simulink model "DynamicsHIL"  (R2026a)
settings: Solver=ode4  StopTime=inf  FixedStep=SampleTime
values from neighbouring files (symbols this model uses):
  ArmConstants = struct('l1_dim', l1_dim,                        'l2_dim', l2_dim,                        'Hexa_to_joint_L', L,                        'Mass1', ml1,                        'Mass2', ml2,                        'Inertia1', Hl1,                        'Inertia2', Hl2,                        'MC1', c1,                        'MC2', c2,                        'Servos', Servos)    [init_model.m]    (also in init_var.m)
  HexaConstants = struct('Mass', mb,                         'Inertia', J ,                         'allo', allo,                          'invallo', invallo,                         'kT', kT)    [init_model.m]    (also in init_var.m)
  SampleTime = 0.01    [init_model.m]    (also in px4HostTarget_TCPIP_Read.m = -1)
undefined symbols (not defined in the file or in its folder): Payload
libraries: uavmavlinklib x3, px4MAVLinkBridgelib x2
settings Model: Creator=The MathWorks, Inc.  LastModifiedBy=Carlos Fabian

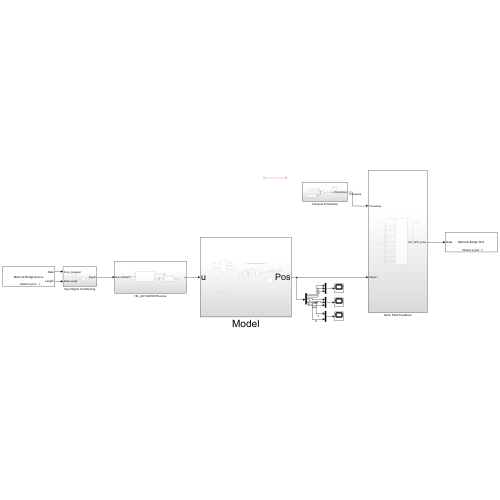
[thumbnail: Simulink's stored preview of the top-level diagram]
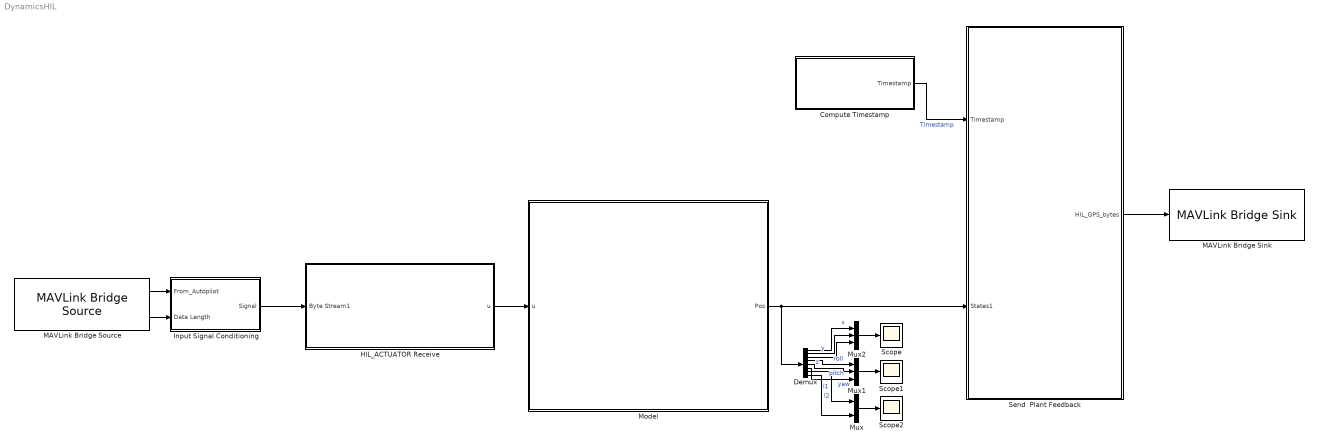
== system DynamicsHIL ==
  Compute Timestamp : Subsystem
  Demux : Demux  Outputs=8
  HIL_ACTUATOR Receive : Subsystem
  Input Signal Conditioning : Subsystem
  MAVLink Bridge Sink : px4MAVLinkBridgelib/MAVLink Bridge Sink  PixhawkSerialPorttemp=<Select a port...>  PixhawkSerialPortManually=COM12  FieldTable={ 'UDP', '127.0.0.1', '14550' }
  MAVLink Bridge Source : px4MAVLinkBridgelib/MAVLink Bridge Source  PixhawkSerialPorttemp=<Select a port...>  PixhawkSerialPortManually=COM12  dataLength=MAVLink_Input_Read_Size  FieldTable={ 'UDP', '127.0.0.1', '14550' }  SampleTime=SampleTime
  Model : Subsystem
  Mux : Mux  Inputs=2
  Mux1 : Mux  Inputs=3
  Mux2 : Mux  Inputs=3
  Scope : Scope
  Scope1 : Scope
  Scope2 : Scope
      settings: DataLoggingVariableName=ScopeData2
  Send  Plant Feedback : Subsystem
  wires:
  ? -> ?
  Input Signal Conditioning/1(Signal) -> HIL_ACTUATOR Receive/1(Byte Stream1)
  MAVLink Bridge Source/1 -> Input Signal Conditioning/1(From_Autopilot)
  MAVLink Bridge Source/2 -> Input Signal Conditioning/2(Data Length)
  Send  Plant Feedback/1(HIL_GPS_bytes) -> MAVLink Bridge Sink/1
  Compute Timestamp/1(Timestamp) -> Send  Plant Feedback/1(Timestamp)  "Timestamp"
  Model/1(Pos) -> Demux/1, Send  Plant Feedback/2(States1)
  HIL_ACTUATOR Receive/1(u) -> Model/1(u)
  Demux/1 -> Mux2/1  "x"
  Demux/2 -> Mux2/2  "y"
  Demux/3 -> Mux2/3  "z"
  Demux/4 -> Mux1/1  "roll"
  Demux/5 -> Mux1/2  "pitch"
  Demux/6 -> Mux1/3  "yaw"
  Demux/8 -> Mux/2  "l2"
  Demux/7 -> Mux/1  "l1"
  Mux2/1 -> Scope/1
  Mux1/1 -> Scope1/1
  Mux/1 -> Scope2/1

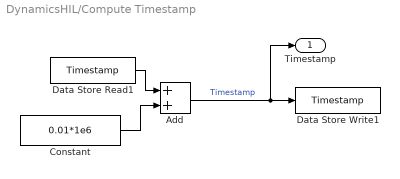
== system DynamicsHIL/Compute Timestamp ==
  Add : Sum
  Constant : Constant  Value=0.01*1e6  OutDataTypeStr=uint64  SampleTime=0.01
  Data Store Read1 : DataStoreRead  DataStoreName=Timestamp  SampleTime=0.01  IndexOptions=Index vector (dialog)  Indices=1  OutputSizes=1
  Data Store Write1 : DataStoreWrite  DataStoreName=Timestamp  SampleTime=0.01  IndexOptions=Index vector (dialog)  Indices=1  OutputSizes=1
  Timestamp : Outport
  wires:
  Data Store Read1/1 -> Add/1
  Add/1 -> Data Store Write1/1, Timestamp/1  "Timestamp"
  Constant/1 -> Add/2

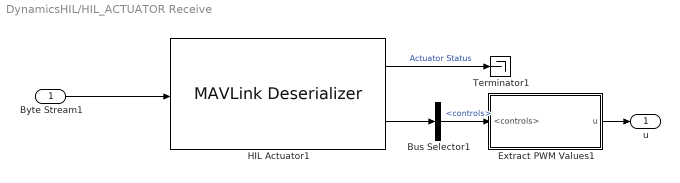
== system DynamicsHIL/HIL_ACTUATOR Receive ==
  Byte Stream1 : Inport
  Bus Selector1 : BusSelector  OutputSignals=Payload.controls
  Extract PWM Values1 : Subsystem
  HIL Actuator1 : uavmavlinklib/MAVLink Deserializer  dialectSource=Specify your own  dialect=common.xml  dialectCustom=C:\Users\Carlos Fabian\Documents\MATLAB\mavlink_custom\uam.xml  version=2  messageType=HIL_ACTUATOR_CONTROLS  inputDataLength=off  SystemIDFilter=off  systemID=1  ComponentIDFilter=off  componentID=1  queueMsg=off  queueMsgSize=50  dropNum=off
  Terminator1 : Terminator
  u : Outport
  wires:
  HIL Actuator1/2 -> Bus Selector1/1
  HIL Actuator1/1 -> Terminator1/1  "Actuator Status"
  Extract PWM Values1/1(u) -> u/1
  Bus Selector1/1 -> Extract PWM Values1/1(<controls>)  "<controls>"
  Byte Stream1/1 -> HIL Actuator1/1

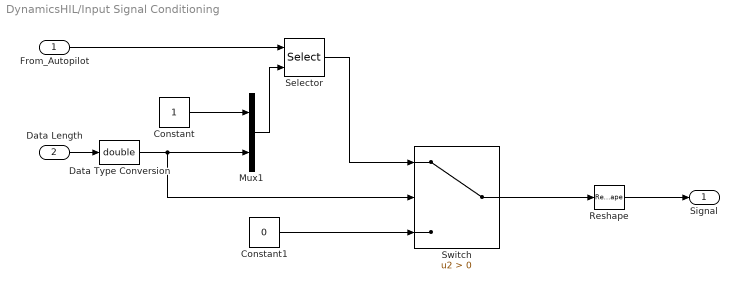
== system DynamicsHIL/Input Signal Conditioning ==
  From_Autopilot : Inport
  Data Length : Inport  Port=2
  Constant : Constant
  Constant1 : Constant  Value=0  OutDataTypeStr=uint8  SampleTime=-1
  Data Type Conversion : DataTypeConversion  OutDataTypeStr=double  SaturateOnIntegerOverflow=off  RndMeth=Floor
  Mux1 : Mux  Inputs=2
  Reshape : Reshape
  Selector : Selector  InputPortWidth=MAVLink_Input_Read_Size  IndexOptions=Starting and ending indices (port)  Indices=[1 3]  OutputSizes=1
  Switch : Switch  Criteria=u2 > Threshold  SaturateOnIntegerOverflow=off  InputSameDT=off
  Signal : Outport
  wires:
  Reshape/1 -> Signal/1
  Mux1/1 -> Selector/2
  Data Length/1 -> Data Type Conversion/1
  Constant/1 -> Mux1/1
  Selector/1 -> Switch/1
  From_Autopilot/1 -> Selector/1
  Constant1/1 -> Switch/3
  Switch/1 -> Reshape/1
  Data Type Conversion/1 -> Switch/2, Mux1/2

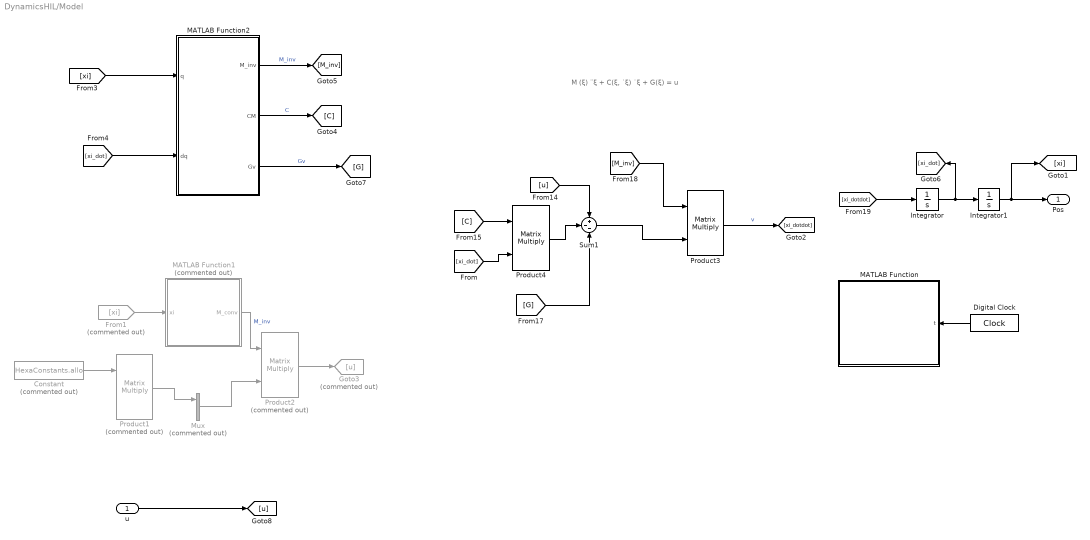
== system DynamicsHIL/Model ==
  note: M (ξ) ¨ξ + C(ξ, ˙ξ) ˙ξ + G(ξ) = u
  u : Inport
  Constant : Constant  Commented=on  Value=HexaConstants.allo
  Digital Clock : DigitalClock  SampleTime=0.01
  From1 : From  Commented=on  GotoTag=xi
  Goto3 : Goto  Commented=on  GotoTag=u
  Integrator : Integrator  InitialCondition=zeros(8,1)
  Integrator1 : Integrator  InitialCondition=zeros(8,1)
  MATLAB Function : MATLAB Function  TreatAsAtomicUnit=on
  MATLAB Function1 : MATLAB Function  Commented=on  TreatAsAtomicUnit=on
  MATLAB Function2 : MATLAB Function  TreatAsAtomicUnit=on
  Mux : Mux  Commented=on  Inputs=2
  Product1 : Product  Commented=on  Multiplication=Matrix(*)
  Product2 : Product  Commented=on  Multiplication=Matrix(*)
  Product3 : Product  Multiplication=Matrix(*)
  Product4 : Product  Multiplication=Matrix(*)
  Sum1 : Sum  Inputs=+--
  Pos : Outport  SampleTime=0.01
  wires:
  Integrator1/1 -> [xi], Pos/1
  [u] -> Sum1/1
  [C] -> Product4/1
  [G] -> Sum1/3
  Sum1/1 -> Product3/2
  [M_inv] -> Product3/1
  Product4/1 -> Sum1/2
  Product3/1 -> [xi_dotdot]  "v"
  [xi_dotdot] -> Integrator/1
  Integrator/1 -> [xi_dot], Integrator1/1
  Digital Clock/1 -> MATLAB Function/1(t)
  MATLAB Function2/3(Gv) -> [G]  "Gv"
  MATLAB Function2/2(CM) -> [C]  "C"
  MATLAB Function2/1(M_inv) -> [M_inv]  "M_inv"
  [xi] -> MATLAB Function2/1(q)
  [xi_dot] -> MATLAB Function2/2(dq)
  [xi_dot] -> Product4/2
  u/1 -> [u]
  Constant/1 -> Product1/1
  Product1/1 -> Mux/1
  Mux/1 -> Product2/2
  Product2/1 -> Goto3/1
  MATLAB Function1/1(M_conv) -> Product2/1  "M_inv"
  From1/1 -> MATLAB Function1/1(xi)

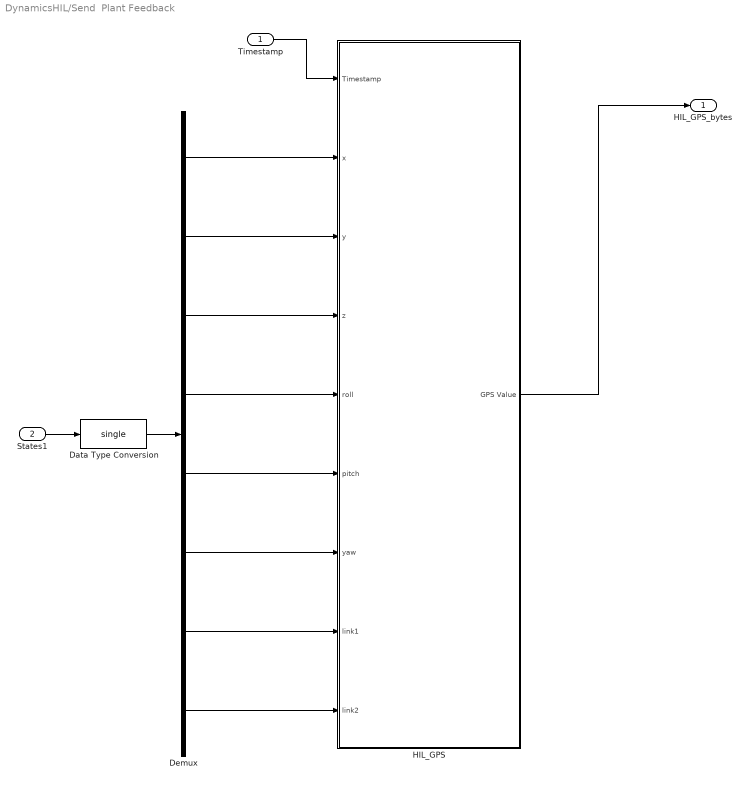
== system DynamicsHIL/Send  Plant Feedback ==
  Timestamp : Inport
  States1 : Inport  Port=2
  Data Type Conversion : DataTypeConversion  OutDataTypeStr=single  SaturateOnIntegerOverflow=off  RndMeth=Floor
  Demux : Demux  Outputs=8
  HIL_GPS : Subsystem
  HIL_GPS_bytes : Outport
  wires:
  Timestamp/1 -> HIL_GPS/1(Timestamp)
  HIL_GPS/1(GPS Value) -> HIL_GPS_bytes/1
  States1/1 -> Data Type Conversion/1
  Demux/1 -> HIL_GPS/2(x)
  Demux/2 -> HIL_GPS/3(y)
  Demux/3 -> HIL_GPS/4(z)
  Demux/4 -> HIL_GPS/5(roll)
  Demux/5 -> HIL_GPS/6(pitch)
  Demux/6 -> HIL_GPS/7(yaw)
  Demux/7 -> HIL_GPS/8(link1)
  Demux/8 -> HIL_GPS/9(link2)
  Data Type Conversion/1 -> Demux/1

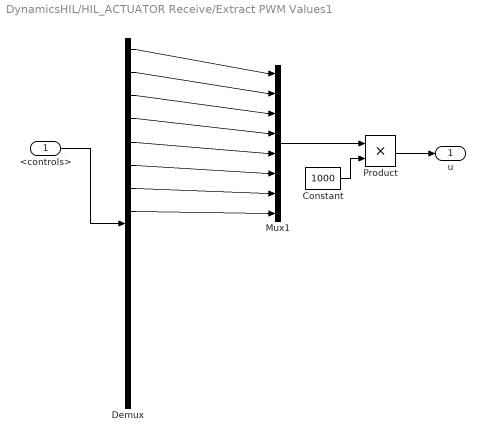
== system DynamicsHIL/HIL_ACTUATOR Receive/Extract PWM Values1 ==
  <controls> : Inport
  Constant : Constant  Value=1000
  Demux : Demux  Outputs=16
  Mux1 : Mux  Inputs=8
  Product : Product
  u : Outport
  wires:
  <controls>/1 -> Demux/1
  Product/1 -> u/1
  Mux1/1 -> Product/1
  Constant/1 -> Product/2
  Demux/1 -> Mux1/1
  Demux/2 -> Mux1/2
  Demux/3 -> Mux1/3
  Demux/4 -> Mux1/4
  Demux/5 -> Mux1/5
  Demux/6 -> Mux1/6
  Demux/7 -> Mux1/7
  Demux/8 -> Mux1/8

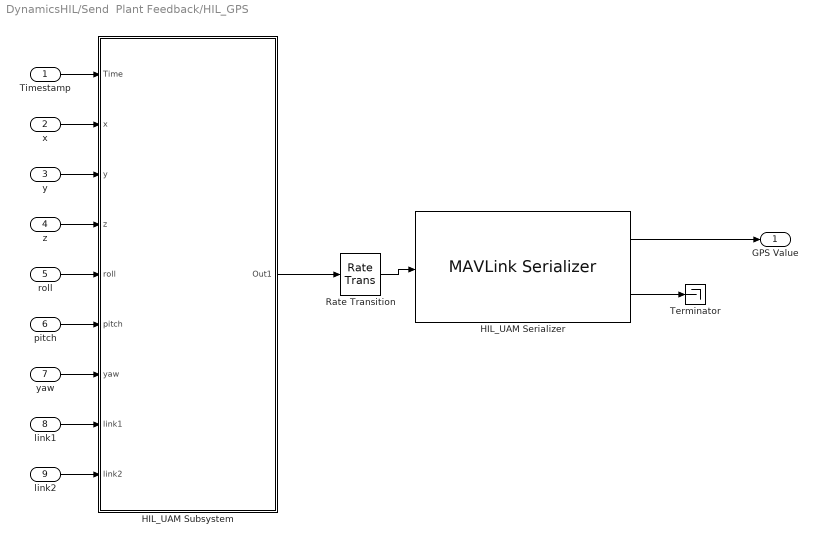
== system DynamicsHIL/Send  Plant Feedback/HIL_GPS ==
  Timestamp : Inport
  x : Inport  Port=2
  y : Inport  Port=3
  z : Inport  Port=4
  roll : Inport  Port=5
  pitch : Inport  Port=6
  yaw : Inport  Port=7
  link1 : Inport  Port=8
  link2 : Inport  Port=9
  HIL_UAM Serializer : uavmavlinklib/MAVLink Serializer  dialectSource=Specify your own  dialect=common.xml  dialectCustom=C:\Users\Carlos Fabian\Documents\MATLAB\UAM_Hexa_PID\mavlink_custom\common.xml  version=2  messageType=UAM_STATES
  HIL_UAM Subsystem : Subsystem
  Rate Transition : RateTransition  OutPortSampleTime=0.01
  Terminator : Terminator
  GPS Value : Outport
  wires:
  Timestamp/1 -> HIL_UAM Subsystem/1(Time)
  x/1 -> HIL_UAM Subsystem/2(x)
  y/1 -> HIL_UAM Subsystem/3(y)
  z/1 -> HIL_UAM Subsystem/4(z)
  yaw/1 -> HIL_UAM Subsystem/7(yaw)
  pitch/1 -> HIL_UAM Subsystem/6(pitch)
  roll/1 -> HIL_UAM Subsystem/5(roll)
  link2/1 -> HIL_UAM Subsystem/9(link2)
  link1/1 -> HIL_UAM Subsystem/8(link1)
  HIL_UAM Subsystem/1(Out1) -> Rate Transition/1
  HIL_UAM Serializer/2 -> Terminator/1
  HIL_UAM Serializer/1 -> GPS Value/1
  Rate Transition/1 -> HIL_UAM Serializer/1

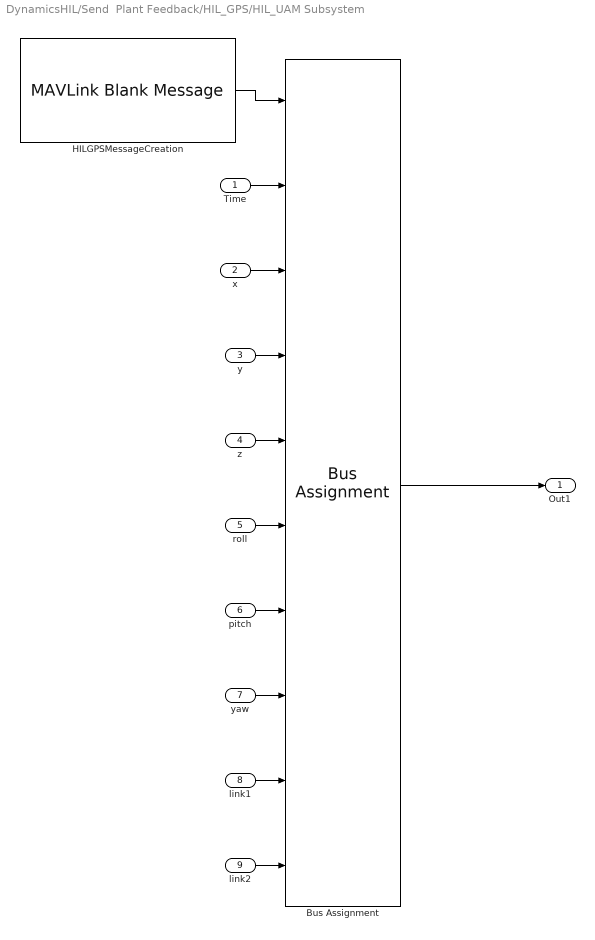
== system DynamicsHIL/Send  Plant Feedback/HIL_GPS/HIL_UAM Subsystem ==
  Time : Inport
  x : Inport  Port=2
  y : Inport  Port=3
  z : Inport  Port=4
  roll : Inport  Port=5
  pitch : Inport  Port=6
  yaw : Inport  Port=7
  link1 : Inport  Port=8
  link2 : Inport  Port=9
  Bus Assignment : BusAssignment  AssignedSignals=Payload.time_usec,Payload.pos_x,Payload.pos_y,Payload.pos_z,Payload.roll,Payload.pitch,Payload.yaw,Payload.link_one,Payload.link_two
  HILGPSMessageCreation : uavmavlinklib/MAVLink Blank Message  dialectSource=Specify your own  dialect=common.xml  dialectCustom=C:\Users\Carlos Fabian\Documents\MATLAB\UAM_Hexa_PID\mavlink_custom\common.xml  version=2  messageType=UAM_STATES  SystemID=2  ComponentID=51  SampleTime=0.01
  Out1 : Outport
  wires:
  HILGPSMessageCreation/1 -> Bus Assignment/1
  Bus Assignment/1 -> Out1/1
  Time/1 -> Bus Assignment/2
  roll/1 -> Bus Assignment/6
  yaw/1 -> Bus Assignment/8
  pitch/1 -> Bus Assignment/7
  x/1 -> Bus Assignment/3
  y/1 -> Bus Assignment/4
  z/1 -> Bus Assignment/5
  link1/1 -> Bus Assignment/9
  link2/1 -> Bus Assignment/10

== matlab function DynamicsHIL/Model/MATLAB Function1 ==
  data: xi input; M_conv output
function M_conv  = Get_DCG_Hexa(xi)

phi = xi(4);
theta = xi(5);
psi = xi(6);

C_phi = cos(phi);
S_phi = sin(phi);
    
C_theta = cos(theta);
S_theta = sin(theta);
    
C_psi = cos(psi);
S_psi = sin(psi);

Rb = [
C_psi*C_theta,  C_psi*S_phi*S_theta - C_phi*S_psi,  S_phi*S_psi + C_phi*C_psi*S_theta;
C_theta*S_psi,  C_phi*C_psi + S_psi*S_theta*S_phi, -C_psi*S_phi + S_psi*S_theta*C_phi;
-S_theta,        C_theta*S_phi,                      S_theta*C_phi
];

W = [
1,       0,        -S_theta;
0,   C_phi,  C_theta*S_phi;
0,  -S_phi,  C_theta*C_phi
];

w_inv = inv(W);

M_conv = [Rb, zeros(3,3), zeros(3,2);
    zeros(3,3), w_inv, zeros(3,2);
    zeros(2,3), zeros(2,3), eye(2)];

end

== matlab function DynamicsHIL/Model/MATLAB Function2 ==
  data: q input; dq input; HexaConstants parameter; M_inv output; CM output; Gv output; ArmConstants parameter
function [M_inv, CM, Gv] = Get_DCG_Hexa(q, dq, HexaConstants, ArmConstants)

DM = DMatrix(q, HexaConstants, ArmConstants);
CM = CMatrix(q, dq, HexaConstants, ArmConstants);
Gv = GVector(q, HexaConstants, ArmConstants);

M_inv = inv(DM);

end

== matlab function DynamicsHIL/Model/MATLAB Function ==
  data: t input; PickObj parameter
function GetPickObj(t, PickObj)

Times = PickObj.Time;

if length(Times) == 2
    cond = t <= Times(1) || t >= Times(2);
else
    cond = t <= Times(1);
end

if ~cond
    m = PickObj.Mass;
    r = PickObj.Radius;
    I1 = 2/5*m*r^2;
    I = diag([I1, I1, I1]);
else
    m = 0;
    I = zeros(3, 3);
end

end
